simulink model "inverter_real_completo"  (R2026b)
settings: Solver=VariableStepAuto
values from neighbouring files (symbols this model uses):
  sat_V = sqrt(2/3)*V_slMAX    [coeficientes.m]
settings Model: Creator=lamun  LastModifiedBy=lamun

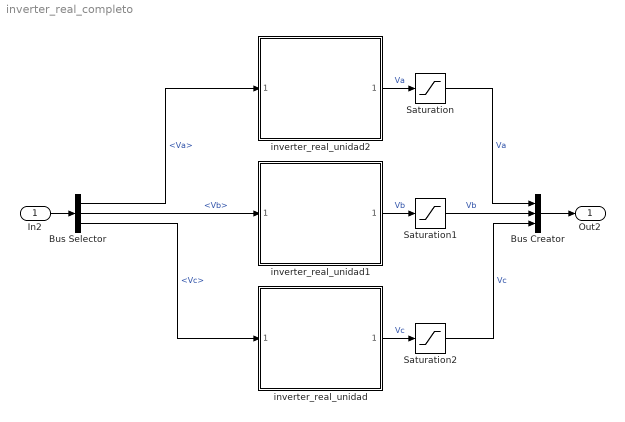
== system inverter_real_completo ==
  In2 : Inport
  Bus Creator : BusCreator  Inputs=3
  Bus Selector : BusSelector  OutputSignals=Va,Vb,Vc
  Saturation : Saturate  UpperLimit=sat_V  LowerLimit=-sat_V
  Saturation1 : Saturate  UpperLimit=sat_V  LowerLimit=-sat_V
  Saturation2 : Saturate  UpperLimit=sat_V  LowerLimit=-sat_V
  inverter_real_unidad : Subsystem  ReferencedSubsystem=inverter_real_unidad
  inverter_real_unidad1 : Subsystem  ReferencedSubsystem=inverter_real_unidad
  inverter_real_unidad2 : Subsystem  ReferencedSubsystem=inverter_real_unidad
  Out2 : Outport
  wires:
  In2/1 -> Bus Selector/1
  Bus Creator/1 -> Out2/1
  Bus Selector/1 -> inverter_real_unidad2/1  "<Va>"
  Bus Selector/2 -> inverter_real_unidad1/1  "<Vb>"
  Bus Selector/3 -> inverter_real_unidad/1  "<Vc>"
  inverter_real_unidad2/1 -> Saturation/1  "Va"
  Saturation/1 -> Bus Creator/1  "Va"
  inverter_real_unidad1/1 -> Saturation1/1  "Vb"
  Saturation1/1 -> Bus Creator/2  "Vb"
  inverter_real_unidad/1 -> Saturation2/1  "Vc"
  Saturation2/1 -> Bus Creator/3  "Vc"
